simulink model "FMS"  (R2018b)
settings: configuration reference "fms_config" (kept outside this file)
values from neighbouring files (symbols this model uses):
  FMS_EXPORT = Simulink.Parameter(FMS_EXPORT_VALUE)    [fms_model_init.m]
  FMS_PARAM = Simulink.Parameter(FMS_PARAM_VALUE)    [fms_model_init.m]
undefined symbols (not defined in the file or in its folder): actuator_cmd, ay_cmd, cmd_mask, ControlMode, ctrl_mode, DiscIntNeverNeededParam, FMS_Cmd, mode, PilotMode, r_cmd, reset, state, status, theta_cmd, timestamp, u_cmd, VehicleState, VehicleStatus, w_cmd, wp_consume, wp_current
libraries: simulink x27, FMT_Model_Lib x21, hdlsllib x4
(part 2 of 3)

== system FMS/FMS Commander/Commander/Arm/Assist/Position/Altitude Command/Detect Movement ==
  FMS_In : Inport
  Abs : Abs
  Abs1 : Abs
  Bus Selector : BusSelector  OutputSignals=Pilot_Cmd.stick_throttle,INS_Out.vd
  Compare To Constant : simulink/Logic and Bit Operations/Compare To Constant  relop=>  const=FMS_PARAM.THROTTLE_DZ  OutDataTypeStr=boolean
  Motion Status : Stateflow chart  TreatAsAtomicUnit=on
  motion_state : Outport
  wires:
  FMS_In/1 -> Bus Selector/1
  Abs1/1 -> Compare To Constant/1
  Motion Status/1(state) -> motion_state/1
  Compare To Constant/1 -> Motion Status/1(motion_req)
  Abs/1 -> Motion Status/2(speed)
  Bus Selector/1 -> Abs1/1  "<stick_throttle>"
  Bus Selector/2 -> Abs/1  "<vd>"

== system FMS/FMS Commander/Commander/Arm/Assist/Position/Heading Command/DeadZone2 ==
  u : Inport
  Dead Zone : DeadZone  LowerValue=-th  UpperValue=th  SaturateOnIntegerOverflow=on
  Gain : Gain  Gain=1/(1-th)
  y : Outport
  wires:
  u/1 -> Dead Zone/1
  Dead Zone/1 -> Gain/1
  Gain/1 -> y/1

== system FMS/FMS Commander/Commander/Arm/Assist/Position/Speed Command/Controller ==
  motion_state : Inport
  In Bus Element : Inport  Port=2  PortName=FMS_In
  In Bus Element1 : Inport  Port=2  PortName=FMS_In
  Brake Control : Subsystem  TreatAsAtomicUnit=on
  Hold Control : Subsystem  TreatAsAtomicUnit=on
  Merge : Merge  Inputs=3
  Move Control : Subsystem  TreatAsAtomicUnit=on
  Saturation1 : Saturate  UpperLimit=FMS_PARAM.VEL_X_LIM  LowerLimit=-FMS_PARAM.VEL_X_LIM
  Switch Case : SwitchCase  CaseConditions={MotionState.Hold, MotionState.Brake, MotionState.Move}  ShowDefaultCase=off
  uv_cmd_mPs : Outport
  wires:
  Move Control/1(uv_cmd_mPs) -> Merge/3
  Brake Control/1(u_cmd_mPs) -> Merge/2
  Hold Control/1(u_cmd_mPs) -> Merge/1
  In Bus Element/1 -> Hold Control/1(FMS_In)
  Switch Case/3 -> Move Control/Action
  Switch Case/2 -> Brake Control/Action
  Switch Case/1 -> Hold Control/Action
  motion_state/1 -> Switch Case/1
  Saturation1/1 -> uv_cmd_mPs/1
  Merge/1 -> Saturation1/1
  In Bus Element1/1 -> Move Control/1(FMS_In)

== system FMS/FMS Commander/Commander/Arm/Assist/Position/Speed Command/Detect Movement ==
  FMS_In : Inport
  Abs2 : Abs
  Bus Selector1 : BusSelector  OutputSignals=Pilot_Cmd.stick_pitch,INS_Out
  Bus_Select : Subsystem
  Compare To Constant1 : simulink/Logic and Bit Operations/Compare To Constant  relop=>  const=FMS_PARAM.PITCH_DZ  OutDataTypeStr=boolean
  Motion State : Stateflow chart  TreatAsAtomicUnit=on
  motion_state : Outport
  wires:
  FMS_In/1 -> Bus Selector1/1
  Compare To Constant1/1 -> Motion State/1(motion_req)
  Abs2/1 -> Compare To Constant1/1
  Motion State/1(state) -> motion_state/1  "pos_ms"
  Bus_Select/1(u_est_B_mPs) -> Motion State/2(speed)
  Bus Selector1/1 -> Abs2/1  "<stick_pitch>"
  Bus Selector1/2 -> Bus_Select/1(INS_Out)  "<INS_Out>"

== system FMS/FMS Commander/Commander/Arm/Assist/Stabilize/Altitude Command /DeadZone2 ==
  u : Inport
  Dead Zone : DeadZone  LowerValue=-th  UpperValue=th  SaturateOnIntegerOverflow=on
  Gain : Gain  Gain=1/(1-th)
  y : Outport
  wires:
  u/1 -> Dead Zone/1
  Dead Zone/1 -> Gain/1
  Gain/1 -> y/1

== system FMS/FMS Commander/Commander/Arm/Assist/Stabilize/Heading Command/DeadZone2 ==
  u : Inport
  Dead Zone : DeadZone  LowerValue=-th  UpperValue=th  SaturateOnIntegerOverflow=on
  Gain : Gain  Gain=1/(1-th)
  y : Outport
  wires:
  u/1 -> Dead Zone/1
  Dead Zone/1 -> Gain/1
  Gain/1 -> y/1

== system FMS/FMS Commander/Commander/Arm/Assist/Stabilize/Speed Command/DeadZone2 ==
  u : Inport
  Dead Zone : DeadZone  LowerValue=-th  UpperValue=th  SaturateOnIntegerOverflow=on
  Gain : Gain  Gain=1/(1-th)
  y : Outport
  wires:
  u/1 -> Dead Zone/1
  Dead Zone/1 -> Gain/1
  Gain/1 -> y/1

== system FMS/FMS Commander/Commander/Arm/Auto/Mission/Mission_SubSystem/Altitude Control ==
  FMS_In : Inport
  Bus Selector3 : BusSelector  OutputSignals=INS_Out.h_R
  Gain : Gain  Gain=FMS_PARAM.Z_P
  Saturation1 : Saturate  UpperLimit=FMS_PARAM.VEL_Z_LIM  LowerLimit=-FMS_PARAM.VEL_Z_LIM
  Sum2 : Sum  Inputs=|+-
  Target Height : Subsystem
  w_cmd_mPs : Outport
  wires:
  FMS_In/1 -> Bus Selector3/1, Target Height/1(FMS_In)
  Bus Selector3/1 -> Sum2/1  "<h_R>"
  Sum2/1 -> Gain/1
  Gain/1 -> Saturation1/1
  Target Height/1(h_R_sp) -> Sum2/2  "h_R_sp"
  Saturation1/1 -> w_cmd_mPs/1

== system FMS/FMS Commander/Commander/Arm/Auto/Mission/Mission_SubSystem/Position Command ==
  FMS_In : Inport
  L1 : Constant  Value=FMS_PARAM.L1  OutDataTypeStr=single
  Velocity Commander : Subsystem
  Way Points : Subsystem
  r_cmd : Outport
  wires:
  FMS_In/1 -> Velocity Commander/5(FMS_In), Way Points/1(FMS_In)
  Way Points/3(p3) -> Velocity Commander/3(p3)
  Velocity Commander/1(r_cmd) -> r_cmd/1
  Way Points/1(p1) -> Velocity Commander/1(p1)
  L1/1 -> Velocity Commander/4(L1)
  Way Points/2(p2) -> Velocity Commander/2(p2)

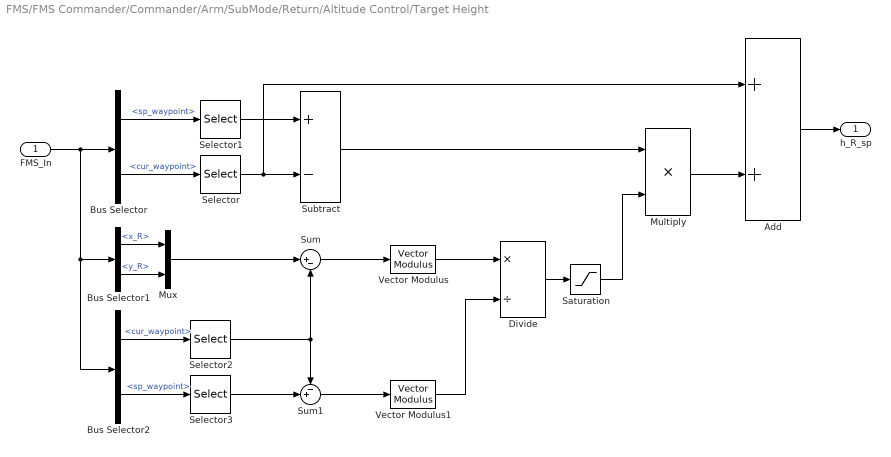
== system FMS/FMS Commander/Commander/Arm/SubMode/Return/Altitude Control/Target Height ==
  FMS_In : Inport
  Add : Sum
  Bus Selector : BusSelector  OutputSignals=Cmd_In.sp_waypoint,Cmd_In.cur_waypoint
  Bus Selector1 : BusSelector  OutputSignals=INS_Out.x_R,INS_Out.y_R
  Bus Selector2 : BusSelector  OutputSignals=Cmd_In.cur_waypoint,Cmd_In.sp_waypoint
  Divide : Product  Inputs=*/
  Multiply : Product
  Mux : Mux  Inputs=2
  Saturation : Saturate  UpperLimit=1  LowerLimit=0
  Selector : Selector  InputPortWidth=3  IndexOptions=Index vector (dialog)  Indices=3  OutputSizes=1
  Selector1 : Selector  InputPortWidth=3  IndexOptions=Index vector (dialog)  Indices=3  OutputSizes=1
  Selector2 : Selector  InputPortWidth=3  IndexOptions=Index vector (dialog)  Indices=[1 2]  OutputSizes=1
  Selector3 : Selector  InputPortWidth=3  IndexOptions=Index vector (dialog)  Indices=[1 2]  OutputSizes=1
  Subtract : Sum  Inputs=+-
  Sum : Sum  Inputs=|+-
  Sum1 : Sum  Inputs=-+|
  Vector Modulus : FMT_Model_Lib/Math/Vector Modulus
      settings: SourceProductName=FMT Toolbox
  Vector Modulus1 : FMT_Model_Lib/Math/Vector Modulus
      settings: SourceProductName=FMT Toolbox
  h_R_sp : Outport
  wires:
  Multiply/1 -> Add/2
  Bus Selector1/1 -> Mux/1  "<x_R>"
  Bus Selector/1 -> Selector1/1  "<sp_waypoint>"
  Vector Modulus1/1 -> Divide/2
  Sum1/1 -> Vector Modulus1/1
  Sum/1 -> Vector Modulus/1
  Selector2/1 -> Sum1/1, Sum/2
  FMS_In/1 -> Bus Selector2/1, Bus Selector1/1, Bus Selector/1
  Bus Selector2/2 -> Selector3/1  "<sp_waypoint>"
  Vector Modulus/1 -> Divide/1
  Bus Selector1/2 -> Mux/2  "<y_R>"
  Bus Selector2/1 -> Selector2/1  "<cur_waypoint>"
  Selector1/1 -> Subtract/1
  Mux/1 -> Sum/1
  Subtract/1 -> Multiply/1
  Divide/1 -> Saturation/1
  Selector3/1 -> Sum1/2
  Bus Selector/2 -> Selector/1  "<cur_waypoint>"
  Selector/1 -> Add/1, Subtract/2
  Saturation/1 -> Multiply/2
  Add/1 -> h_R_sp/1

== system FMS/FMS Commander/Commander/Arm/SubMode/Return/Position Command/Velocity Commander ==
  p1 : Inport
  p2 : Inport  Port=2
  p3 : Inport  Port=3
  L1 : Inport  Port=4
  In Bus Element : Inport  Port=5  PortName=FMS_In  Element=INS_Out.vn
  In Bus Element1 : Inport  Port=5  PortName=FMS_In  Element=INS_Out.ve
  AccToRate : Gain  Gain=FMS_PARAM.ACC2RATE
  L1 Reference WP : Subsystem
  Lateral Acceleration : Subsystem
  Mux1 : Mux  Inputs=2
  r_cmd : Outport
  wires:
  p3/1 -> Lateral Acceleration/3(p3), L1 Reference WP/3(P3)
  In Bus Element1/1 -> Mux1/2
  Mux1/1 -> Lateral Acceleration/1(Vg)
  p2/1 -> L1 Reference WP/2(P2)
  Lateral Acceleration/1(l1_a_cmd) -> AccToRate/1
  In Bus Element/1 -> Mux1/1
  L1 Reference WP/1(L1_WP) -> Lateral Acceleration/2(L1_WP)  "L1_WP"
  p1/1 -> L1 Reference WP/1(P1)
  L1/1 -> L1 Reference WP/4(L1), Lateral Acceleration/4(L1)
  AccToRate/1 -> r_cmd/1

== system FMS/FMS Commander/Commander/Arm/SubMode/Return/Position Command/Way Points ==
  note: P1: path start point
      | P2: path end point
      | P3: vehicle point
  FMS_In : Inport
  Bus Selector : BusSelector  OutputSignals=INS_Out.x_R,INS_Out.y_R
  Bus Selector1 : BusSelector  OutputSignals=Cmd_In.sp_waypoint
  Bus Selector2 : BusSelector  OutputSignals=Cmd_In.cur_waypoint
  Mux : Mux  Inputs=2
  Reshape : Reshape  OutputDimensionality=Customize  OutputDimensions=[2,1]
  Reshape1 : Reshape  OutputDimensionality=Customize  OutputDimensions=[2,1]
  Reshape2 : Reshape  OutputDimensionality=Customize  OutputDimensions=[2,1]
  Selector : Selector  InputPortWidth=3  IndexOptions=Index vector (dialog)  Indices=[1 2]  OutputSizes=1
  Selector1 : Selector  InputPortWidth=3  IndexOptions=Index vector (dialog)  Indices=[1 2]  OutputSizes=1
  p1 : Outport
  p2 : Outport  Port=2
  p3 : Outport  Port=3
  wires:
  Reshape2/1 -> p3/1
  Reshape1/1 -> p1/1
  Reshape/1 -> p2/1
  Bus Selector/2 -> Mux/2  "<y_R>"
  Bus Selector/1 -> Mux/1  "<x_R>"
  Mux/1 -> Reshape2/1
  FMS_In/1 -> Bus Selector2/1, Bus Selector1/1, Bus Selector/1
  Bus Selector1/1 -> Selector/1  "<sp_waypoint>"
  Selector/1 -> Reshape/1
  Bus Selector2/1 -> Selector1/1  "<cur_waypoint>"
  Selector1/1 -> Reshape1/1

== system FMS/FMS Commander/Commander/Arm/Assist/Altitude/Altitude Command/Controller/Brake Control ==
  Action Port : ActionPort  InitializeStates=reset  ActionType=case
  Brake Speed : Constant  Value=0  VectorParams1D=off  OutDataTypeStr=single
  w_cmd_mPs : Outport
  wires:
  Brake Speed/1 -> w_cmd_mPs/1

== system FMS/FMS Commander/Commander/Arm/Assist/Altitude/Altitude Command/Controller/Hold Control ==
  FMS_In : Inport
  Action Port : ActionPort  InitializeStates=reset  ActionType=case
  Bus_Selection : Subsystem
  Delay : Delay  DelayLength=1  InitialConditionSource=Input port
      settings: InputPortMap=u0,p4
  Gain2 : Gain  Gain=FMS_PARAM.Z_P  OutDataTypeStr=single
  Sum : Sum  Inputs=-+|
  w_cmd_mPs : Outport
  wires:
  FMS_In/1 -> Bus_Selection/1(FMS_In)
  Delay/1 -> Sum/2, Delay/1  "z_cmd_R"
  Sum/1 -> Gain2/1  "z_err_R"
  Bus_Selection/1(z_R_m) -> Delay/2, Sum/1  "z_est_R"
  Gain2/1 -> w_cmd_mPs/1

== system FMS/FMS Commander/Commander/Arm/Assist/Altitude/Altitude Command/Controller/Move Control ==
  FMS_In : Inport
  Action Port : ActionPort  InitializeStates=reset  ActionType=case
  Bus Selector : BusSelector  OutputSignals=Pilot_Cmd.stick_throttle
  DeadZone : Subsystem  mask{th=FMS_PARAM.THROTTLE_DZ}
      mask prompts: th "Threshold"
      mask Display: disp('Dead Zone')
  Gain1 : Gain  Gain=-FMS_PARAM.VEL_Z_LIM  OutDataTypeStr=single
  w_cmd_mPs : Outport
  wires:
  DeadZone/1(y) -> Gain1/1
  Bus Selector/1 -> DeadZone/1(u)  "<stick_throttle>"
  FMS_In/1 -> Bus Selector/1
  Gain1/1 -> w_cmd_mPs/1

== system FMS/FMS Commander/Commander/Arm/Assist/Position/Altitude Command/Controller/Brake Control ==
  Action Port : ActionPort  InitializeStates=reset  ActionType=case
  Brake Speed : Constant  Value=0  VectorParams1D=off  OutDataTypeStr=single
  w_cmd_mPs : Outport
  wires:
  Brake Speed/1 -> w_cmd_mPs/1

== system FMS/FMS Commander/Commander/Arm/Assist/Position/Altitude Command/Controller/Hold Control ==
  FMS_In : Inport
  Action Port : ActionPort  InitializeStates=reset  ActionType=case
  Bus_Selection : Subsystem
  Delay : Delay  DelayLength=1  InitialConditionSource=Input port
      settings: InputPortMap=u0,p4
  Gain2 : Gain  Gain=FMS_PARAM.Z_P  OutDataTypeStr=single
  Sum : Sum  Inputs=-+|
  w_cmd_mPs : Outport
  wires:
  FMS_In/1 -> Bus_Selection/1(FMS_In)
  Delay/1 -> Sum/2, Delay/1  "z_cmd_R"
  Sum/1 -> Gain2/1  "z_err_R"
  Bus_Selection/1(z_R_m) -> Delay/2, Sum/1  "z_est_R"
  Gain2/1 -> w_cmd_mPs/1

== system FMS/FMS Commander/Commander/Arm/Assist/Position/Altitude Command/Controller/Move Control ==
  FMS_In : Inport
  Action Port : ActionPort  InitializeStates=reset  ActionType=case
  Bus Selector : BusSelector  OutputSignals=Pilot_Cmd.stick_throttle
  DeadZone : Subsystem  mask{th=FMS_PARAM.THROTTLE_DZ}
      mask prompts: th "Threshold"
      mask Display: disp('Dead Zone')
  Gain1 : Gain  Gain=-FMS_PARAM.VEL_Z_LIM  OutDataTypeStr=single
  w_cmd_mPs : Outport
  wires:
  DeadZone/1(y) -> Gain1/1
  Bus Selector/1 -> DeadZone/1(u)  "<stick_throttle>"
  FMS_In/1 -> Bus Selector/1
  Gain1/1 -> w_cmd_mPs/1

== system FMS/FMS Commander/Commander/Arm/Assist/Position/Speed Command/Controller/Brake Control ==
  Action Port : ActionPort  InitializeStates=reset  ActionType=case
  Brake Speed : Constant  Value=0  OutDataTypeStr=single
  u_cmd_mPs : Outport
  wires:
  Brake Speed/1 -> u_cmd_mPs/1

== system FMS/FMS Commander/Commander/Arm/Assist/Position/Speed Command/Controller/Hold Control ==
  FMS_In : Inport
  Action Port : ActionPort  InitializeStates=reset  ActionType=case
  Bus Selector : BusSelector  OutputSignals=INS_Out.psi
  Bus_Selection : Subsystem
  Constant : Constant  Value=[0;0]  VectorParams1D=off  OutDataTypeStr=single
  Delay : Delay  DelayLength=1  InitialConditionSource=Input port
      settings: InputPortMap=u0,p4
  Gain2 : Gain  Gain=FMS_PARAM.X_P  OutDataTypeStr=single
  Multiply : Product  Multiplication=Matrix(*)
  Mux : Mux  Inputs=2
  Psi To DCM : FMT_Model_Lib/Transformation/Psi To DCM
      settings: SourceProductName=FMT Toolbox
  Reshape : Reshape  OutputDimensionality=Column vector (2-D)
  Selector : Selector  InputPortWidth=3  IndexOptions=Index vector (dialog)  Indices=1  OutputSizes=1
  Sum : Sum  Inputs=-+|
  u_cmd_mPs : Outport
  wires:
  Bus Selector/1 -> Psi To DCM/1  "<psi>"
  Selector/1 -> Gain2/1
  Mux/1 -> Reshape/1
  Multiply/1 -> Selector/1
  Psi To DCM/1 -> Multiply/1  "M_CO"
  Constant/1 -> Mux/2
  FMS_In/1 -> Bus_Selection/1(FMS_In), Bus Selector/1
  Delay/1 -> Sum/2, Delay/1  "x_cmd_R"
  Sum/1 -> Mux/1  "x_err_R"
  Bus_Selection/1(x_R_O_m) -> Delay/2, Sum/1  "x_est_R"
  Gain2/1 -> u_cmd_mPs/1
  Reshape/1 -> Multiply/2

== system FMS/FMS Commander/Commander/Arm/Assist/Position/Speed Command/Controller/Move Control ==
  FMS_In : Inport
  Action Port : ActionPort  InitializeStates=reset  ActionType=case
  Bus Selector : BusSelector  OutputSignals=Pilot_Cmd.stick_pitch
  DeadZone : Subsystem  mask{th=FMS_PARAM.PITCH_DZ}
      mask prompts: th "Threshold"
      mask Display: disp('Dead Zone')
  Gain6 : Gain  Gain=FMS_PARAM.VEL_X_LIM  OutDataTypeStr=single
  uv_cmd_mPs : Outport
  wires:
  Gain6/1 -> uv_cmd_mPs/1
  FMS_In/1 -> Bus Selector/1
  Bus Selector/1 -> DeadZone/1(u)  "<stick_pitch>"
  DeadZone/1(y) -> Gain6/1

== system FMS/FMS Commander/Commander/Arm/Assist/Position/Speed Command/Detect Movement/Bus_Select ==
  INS_Out : Inport
  Bus Selector1 : BusSelector  OutputSignals=vn,ve,vd
  Bus Selector2 : BusSelector  OutputSignals=quat
  Multiply : Product  Multiplication=Matrix(*)
  Mux2 : Mux  Inputs=3
  Quaternion To DCM : FMT_Model_Lib/Quaternion/Quaternion To DCM
      settings: SourceProductName=FMT Toolbox
  Selector : Selector  InputPortWidth=3  IndexOptions=Index vector (dialog)  Indices=1  OutputSizes=1
  u_est_B_mPs : Outport
  wires:
  Quaternion To DCM/1 -> Multiply/1
  Bus Selector2/1 -> Quaternion To DCM/1  "<quat>"
  Mux2/1 -> Multiply/2
  Bus Selector1/2 -> Mux2/2  "<ve>"
  Bus Selector1/1 -> Mux2/1  "<vn>"
  INS_Out/1 -> Bus Selector2/1, Bus Selector1/1
  Multiply/1 -> Selector/1
  Selector/1 -> u_est_B_mPs/1
  Bus Selector1/3 -> Mux2/3  "<vd>"

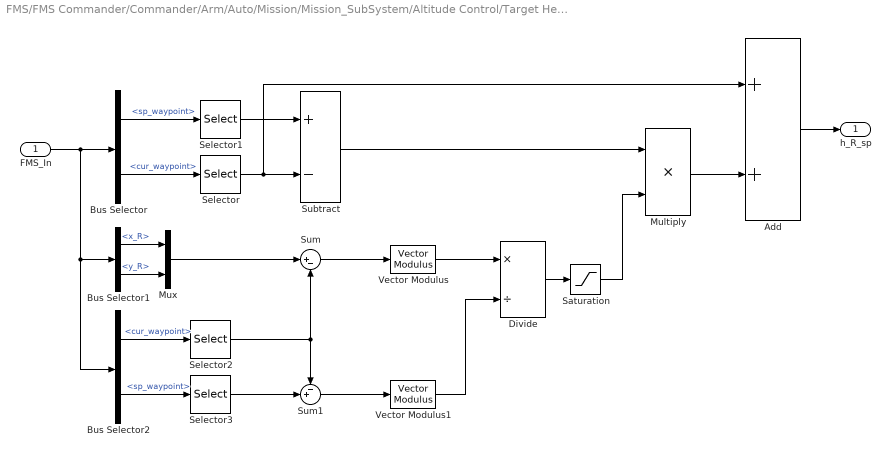
== system FMS/FMS Commander/Commander/Arm/Auto/Mission/Mission_SubSystem/Altitude Control/Target Height ==
  FMS_In : Inport
  Add : Sum
  Bus Selector : BusSelector  OutputSignals=Cmd_In.sp_waypoint,Cmd_In.cur_waypoint
  Bus Selector1 : BusSelector  OutputSignals=INS_Out.x_R,INS_Out.y_R
  Bus Selector2 : BusSelector  OutputSignals=Cmd_In.cur_waypoint,Cmd_In.sp_waypoint
  Divide : Product  Inputs=*/
  Multiply : Product
  Mux : Mux  Inputs=2
  Saturation : Saturate  UpperLimit=1  LowerLimit=0
  Selector : Selector  InputPortWidth=3  IndexOptions=Index vector (dialog)  Indices=3  OutputSizes=1
  Selector1 : Selector  InputPortWidth=3  IndexOptions=Index vector (dialog)  Indices=3  OutputSizes=1
  Selector2 : Selector  InputPortWidth=3  IndexOptions=Index vector (dialog)  Indices=[1 2]  OutputSizes=1
  Selector3 : Selector  InputPortWidth=3  IndexOptions=Index vector (dialog)  Indices=[1 2]  OutputSizes=1
  Subtract : Sum  Inputs=+-
  Sum : Sum  Inputs=|+-
  Sum1 : Sum  Inputs=-+|
  Vector Modulus : FMT_Model_Lib/Math/Vector Modulus
      settings: SourceProductName=FMT Toolbox
  Vector Modulus1 : FMT_Model_Lib/Math/Vector Modulus
      settings: SourceProductName=FMT Toolbox
  h_R_sp : Outport
  wires:
  Multiply/1 -> Add/2
  Bus Selector1/1 -> Mux/1  "<x_R>"
  Bus Selector/1 -> Selector1/1  "<sp_waypoint>"
  Vector Modulus1/1 -> Divide/2
  Sum1/1 -> Vector Modulus1/1
  Sum/1 -> Vector Modulus/1
  Selector2/1 -> Sum1/1, Sum/2
  FMS_In/1 -> Bus Selector2/1, Bus Selector1/1, Bus Selector/1
  Bus Selector2/2 -> Selector3/1  "<sp_waypoint>"
  Vector Modulus/1 -> Divide/1
  Bus Selector1/2 -> Mux/2  "<y_R>"
  Bus Selector2/1 -> Selector2/1  "<cur_waypoint>"
  Selector1/1 -> Subtract/1
  Mux/1 -> Sum/1
  Subtract/1 -> Multiply/1
  Divide/1 -> Saturation/1
  Selector3/1 -> Sum1/2
  Bus Selector/2 -> Selector/1  "<cur_waypoint>"
  Selector/1 -> Add/1, Subtract/2
  Saturation/1 -> Multiply/2
  Add/1 -> h_R_sp/1

== system FMS/FMS Commander/Commander/Arm/Auto/Mission/Mission_SubSystem/Position Command/Velocity Commander ==
  p1 : Inport
  p2 : Inport  Port=2
  p3 : Inport  Port=3
  L1 : Inport  Port=4
  In Bus Element : Inport  Port=5  PortName=FMS_In  Element=INS_Out.vn
  In Bus Element1 : Inport  Port=5  PortName=FMS_In  Element=INS_Out.ve
  AccToRate : Gain  Gain=FMS_PARAM.ACC2RATE
  L1 Reference WP : Subsystem
  Lateral Acceleration : Subsystem
  Mux1 : Mux  Inputs=2
  r_cmd : Outport
  wires:
  p3/1 -> Lateral Acceleration/3(p3), L1 Reference WP/3(P3)
  In Bus Element1/1 -> Mux1/2
  Mux1/1 -> Lateral Acceleration/1(Vg)
  p2/1 -> L1 Reference WP/2(P2)
  Lateral Acceleration/1(l1_a_cmd) -> AccToRate/1
  In Bus Element/1 -> Mux1/1
  L1 Reference WP/1(L1_WP) -> Lateral Acceleration/2(L1_WP)  "L1_WP"
  p1/1 -> L1 Reference WP/1(P1)
  L1/1 -> L1 Reference WP/4(L1), Lateral Acceleration/4(L1)
  AccToRate/1 -> r_cmd/1

== system FMS/FMS Commander/Commander/Arm/Auto/Mission/Mission_SubSystem/Position Command/Way Points ==
  note: P1: path start point
      | P2: path end point
      | P3: vehicle point
  FMS_In : Inport
  Bus Selector : BusSelector  OutputSignals=INS_Out.x_R,INS_Out.y_R
  Bus Selector1 : BusSelector  OutputSignals=Cmd_In.sp_waypoint
  Bus Selector2 : BusSelector  OutputSignals=Cmd_In.cur_waypoint
  Mux : Mux  Inputs=2
  Reshape : Reshape  OutputDimensionality=Customize  OutputDimensions=[2,1]
  Reshape1 : Reshape  OutputDimensionality=Customize  OutputDimensions=[2,1]
  Reshape2 : Reshape  OutputDimensionality=Customize  OutputDimensions=[2,1]
  Selector : Selector  InputPortWidth=3  IndexOptions=Index vector (dialog)  Indices=[1 2]  OutputSizes=1
  Selector1 : Selector  InputPortWidth=3  IndexOptions=Index vector (dialog)  Indices=[1 2]  OutputSizes=1
  p1 : Outport
  p2 : Outport  Port=2
  p3 : Outport  Port=3
  wires:
  Reshape2/1 -> p3/1
  Reshape1/1 -> p1/1
  Reshape/1 -> p2/1
  Bus Selector/2 -> Mux/2  "<y_R>"
  Bus Selector/1 -> Mux/1  "<x_R>"
  Mux/1 -> Reshape2/1
  FMS_In/1 -> Bus Selector2/1, Bus Selector1/1, Bus Selector/1
  Bus Selector1/1 -> Selector/1  "<sp_waypoint>"
  Selector/1 -> Reshape/1
  Bus Selector2/1 -> Selector1/1  "<cur_waypoint>"
  Selector1/1 -> Reshape1/1

== system FMS/FMS Commander/Commander/Arm/SubMode/Return/Position Command/Velocity Commander/L1 Reference WP ==
  P1 : Inport
  P2 : Inport  Port=2
  P3 : Inport  Port=3
  L1 : Inport  Port=4
  Compare To Constant : simulink/Logic and Bit Operations/Compare To Constant  relop=>=  const=0  OutDataTypeStr=boolean
  Compare To Constant1 : simulink/Logic and Bit Operations/Compare To Constant  relop=>  const=0  OutDataTypeStr=boolean
  NearbyRefWP : MATLAB Function  TreatAsAtomicUnit=on
  OutRegionRegWP : MATLAB Function  TreatAsAtomicUnit=on
  Reshape : Reshape  OutputDimensionality=Customize  OutputDimensions=[2,1]
  SearchL1RefWP : MATLAB Function  TreatAsAtomicUnit=on
  Switch : Switch  Criteria=u2 > Threshold
  Switch1 : Switch  Criteria=u2 > Threshold
  L1_WP : Outport
  wires:
  Reshape/1 -> L1_WP/1
  Compare To Constant/1 -> Switch/2
  NearbyRefWP/2(d) -> Compare To Constant1/1  "distance"
  SearchL1RefWP/2(u) -> Compare To Constant/1  "l1_u"
  Compare To Constant1/1 -> Switch1/2
  P1/1 -> SearchL1RefWP/1(P1), OutRegionRegWP/1(P1)
  P2/1 -> SearchL1RefWP/2(P2), NearbyRefWP/1(P2), OutRegionRegWP/2(P2)
  P3/1 -> NearbyRefWP/2(P3), SearchL1RefWP/3(P3), OutRegionRegWP/3(P3)
  Switch/1 -> Switch1/3
  L1/1 -> SearchL1RefWP/4(L1), NearbyRefWP/3(L1)
  OutRegionRegWP/1(P) -> Switch/3  "out_WP"
  Switch1/1 -> Reshape/1
  SearchL1RefWP/1(P) -> Switch/1  "L1_Ref_P"
  NearbyRefWP/1(P) -> Switch1/1  "NearbyWP"

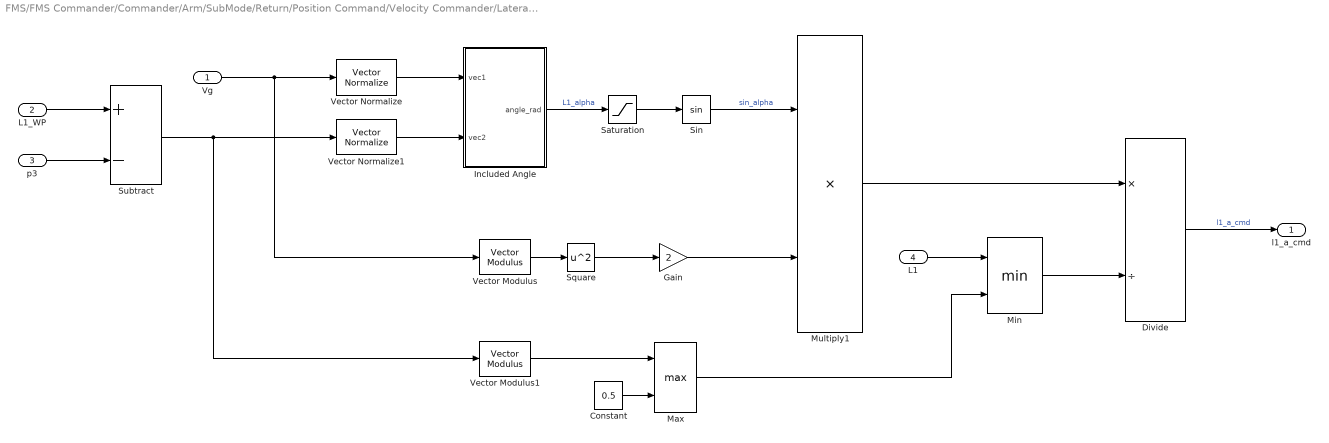
== system FMS/FMS Commander/Commander/Arm/SubMode/Return/Position Command/Velocity Commander/Lateral Acceleration ==
  Vg : Inport
  L1_WP : Inport  Port=2
  p3 : Inport  Port=3
  L1 : Inport  Port=4
  Constant : Constant  Value=0.5  OutDataTypeStr=Inherit: Inherit via back propagation
  Divide : Product  Inputs=*/
  Gain : Gain  Gain=2
  Included Angle : Subsystem
  Max : MinMax  Function=max  Inputs=2
  Min : MinMax  Inputs=2
  Multiply1 : Product
  Saturation : Saturate  UpperLimit=pi/2  LowerLimit=-pi/2
  Sin : Trigonometry
  Square : Math  Operator=square  SaturateOnIntegerOverflow=on
  Subtract : Sum  Inputs=+-
  Vector Modulus : FMT_Model_Lib/Math/Vector Modulus
      settings: SourceProductName=FMT Toolbox
  Vector Modulus1 : FMT_Model_Lib/Math/Vector Modulus
      settings: SourceProductName=FMT Toolbox
  Vector Normalize : FMT_Model_Lib/Math/Vector Normalize
      settings: SourceProductName=FMT Toolbox
  Vector Normalize1 : FMT_Model_Lib/Math/Vector Normalize
      settings: SourceProductName=FMT Toolbox
  l1_a_cmd : Outport
  wires:
  Saturation/1 -> Sin/1
  Included Angle/1(angle_rad) -> Saturation/1  "L1_alpha"
  Vector Modulus/1 -> Square/1
  Subtract/1 -> Vector Modulus1/1, Vector Normalize1/1
  Gain/1 -> Multiply1/2
  L1_WP/1 -> Subtract/1
  Vector Normalize/1 -> Included Angle/1(vec1)
  Multiply1/1 -> Divide/1
  Divide/1 -> l1_a_cmd/1  "l1_a_cmd"
  Vector Normalize1/1 -> Included Angle/2(vec2)
  Square/1 -> Gain/1
  L1/1 -> Min/1
  Vg/1 -> Vector Normalize/1, Vector Modulus/1
  Sin/1 -> Multiply1/1  "sin_alpha"
  p3/1 -> Subtract/2
  Vector Modulus1/1 -> Max/1
  Constant/1 -> Max/2
  Max/1 -> Min/2
  Min/1 -> Divide/2

== system FMS/FMS Commander/Commander/Arm/Assist/Altitude/Altitude Command/Controller/Hold Control/Bus_Selection ==
  FMS_In : Inport
  Bus Selector2 : BusSelector  OutputSignals=INS_Out.h_R
  Gain : Gain  Gain=-1
  z_R_m : Outport
  wires:
  Gain/1 -> z_R_m/1
  Bus Selector2/1 -> Gain/1  "<h_R>"
  FMS_In/1 -> Bus Selector2/1

== system FMS/FMS Commander/Commander/Arm/Assist/Altitude/Altitude Command/Controller/Move Control/DeadZone ==
  u : Inport
  Dead Zone : DeadZone  LowerValue=-th  UpperValue=th  SaturateOnIntegerOverflow=on
  Gain : Gain  Gain=1/(1-th)
  y : Outport
  wires:
  Gain/1 -> y/1
  Dead Zone/1 -> Gain/1
  u/1 -> Dead Zone/1

== system FMS/FMS Commander/Commander/Arm/Assist/Position/Altitude Command/Controller/Hold Control/Bus_Selection ==
  FMS_In : Inport
  Bus Selector2 : BusSelector  OutputSignals=INS_Out.h_R
  Gain : Gain  Gain=-1
  z_R_m : Outport
  wires:
  Gain/1 -> z_R_m/1
  Bus Selector2/1 -> Gain/1  "<h_R>"
  FMS_In/1 -> Bus Selector2/1

== system FMS/FMS Commander/Commander/Arm/Assist/Position/Altitude Command/Controller/Move Control/DeadZone ==
  u : Inport
  Dead Zone : DeadZone  LowerValue=-th  UpperValue=th  SaturateOnIntegerOverflow=on
  Gain : Gain  Gain=1/(1-th)
  y : Outport
  wires:
  Gain/1 -> y/1
  Dead Zone/1 -> Gain/1
  u/1 -> Dead Zone/1

== system FMS/FMS Commander/Commander/Arm/Assist/Position/Speed Command/Controller/Hold Control/Bus_Selection ==
  FMS_In : Inport
  Bus Selector2 : BusSelector  OutputSignals=INS_Out.x_R
  x_R_O_m : Outport
  wires:
  Bus Selector2/1 -> x_R_O_m/1  "<x_R>"
  FMS_In/1 -> Bus Selector2/1

== system FMS/FMS Commander/Commander/Arm/Assist/Position/Speed Command/Controller/Move Control/DeadZone ==
  u : Inport
  Dead Zone : DeadZone  LowerValue=-th  UpperValue=th  SaturateOnIntegerOverflow=on
  Gain : Gain  Gain=1/(1-th)
  y : Outport
  wires:
  Gain/1 -> y/1
  Dead Zone/1 -> Gain/1
  u/1 -> Dead Zone/1

== system FMS/FMS Commander/Commander/Arm/Auto/Mission/Mission_SubSystem/Position Command/Velocity Commander/L1 Reference WP ==
  P1 : Inport
  P2 : Inport  Port=2
  P3 : Inport  Port=3
  L1 : Inport  Port=4
  Compare To Constant : simulink/Logic and Bit Operations/Compare To Constant  relop=>=  const=0  OutDataTypeStr=boolean
  Compare To Constant1 : simulink/Logic and Bit Operations/Compare To Constant  relop=>  const=0  OutDataTypeStr=boolean
  NearbyRefWP : MATLAB Function  TreatAsAtomicUnit=on
  OutRegionRegWP : MATLAB Function  TreatAsAtomicUnit=on
  Reshape : Reshape  OutputDimensionality=Customize  OutputDimensions=[2,1]
  SearchL1RefWP : MATLAB Function  TreatAsAtomicUnit=on
  Switch : Switch  Criteria=u2 > Threshold
  Switch1 : Switch  Criteria=u2 > Threshold
  L1_WP : Outport
  wires:
  Reshape/1 -> L1_WP/1
  Compare To Constant/1 -> Switch/2
  NearbyRefWP/2(d) -> Compare To Constant1/1  "distance"
  SearchL1RefWP/2(u) -> Compare To Constant/1  "l1_u"
  Compare To Constant1/1 -> Switch1/2
  P1/1 -> SearchL1RefWP/1(P1), OutRegionRegWP/1(P1)
  P2/1 -> SearchL1RefWP/2(P2), NearbyRefWP/1(P2), OutRegionRegWP/2(P2)
  P3/1 -> NearbyRefWP/2(P3), SearchL1RefWP/3(P3), OutRegionRegWP/3(P3)
  Switch/1 -> Switch1/3
  L1/1 -> SearchL1RefWP/4(L1), NearbyRefWP/3(L1)
  OutRegionRegWP/1(P) -> Switch/3  "out_WP"
  Switch1/1 -> Reshape/1
  SearchL1RefWP/1(P) -> Switch/1  "L1_Ref_P"
  NearbyRefWP/1(P) -> Switch1/1  "NearbyWP"

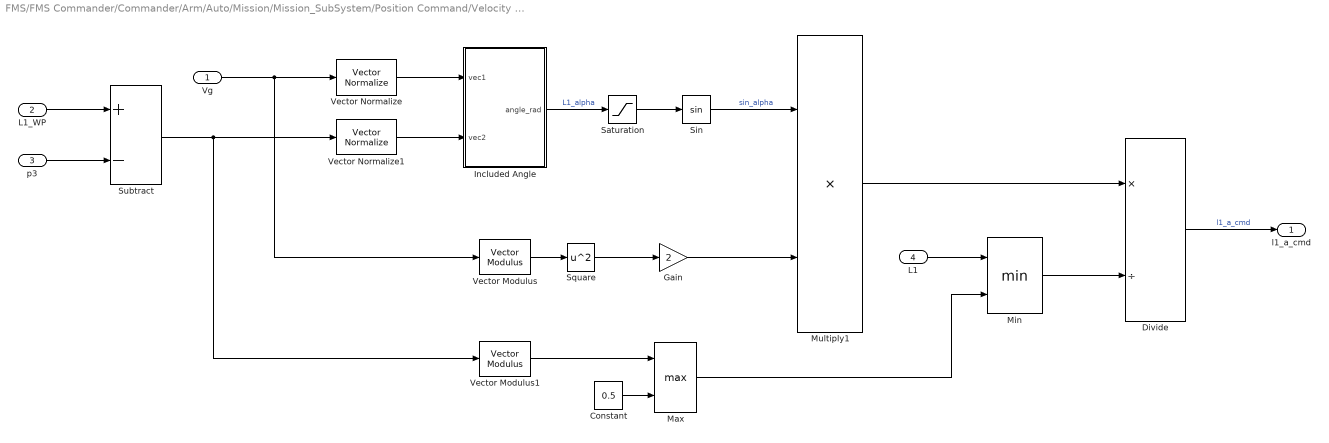
== system FMS/FMS Commander/Commander/Arm/Auto/Mission/Mission_SubSystem/Position Command/Velocity Commander/Lateral Acceleration ==
  Vg : Inport
  L1_WP : Inport  Port=2
  p3 : Inport  Port=3
  L1 : Inport  Port=4
  Constant : Constant  Value=0.5  OutDataTypeStr=Inherit: Inherit via back propagation
  Divide : Product  Inputs=*/
  Gain : Gain  Gain=2
  Included Angle : Subsystem
  Max : MinMax  Function=max  Inputs=2
  Min : MinMax  Inputs=2
  Multiply1 : Product
  Saturation : Saturate  UpperLimit=pi/2  LowerLimit=-pi/2
  Sin : Trigonometry
  Square : Math  Operator=square  SaturateOnIntegerOverflow=on
  Subtract : Sum  Inputs=+-
  Vector Modulus : FMT_Model_Lib/Math/Vector Modulus
      settings: SourceProductName=FMT Toolbox
  Vector Modulus1 : FMT_Model_Lib/Math/Vector Modulus
      settings: SourceProductName=FMT Toolbox
  Vector Normalize : FMT_Model_Lib/Math/Vector Normalize
      settings: SourceProductName=FMT Toolbox
  Vector Normalize1 : FMT_Model_Lib/Math/Vector Normalize
      settings: SourceProductName=FMT Toolbox
  l1_a_cmd : Outport
  wires:
  Saturation/1 -> Sin/1
  Included Angle/1(angle_rad) -> Saturation/1  "L1_alpha"
  Vector Modulus/1 -> Square/1
  Subtract/1 -> Vector Modulus1/1, Vector Normalize1/1
  Gain/1 -> Multiply1/2
  L1_WP/1 -> Subtract/1
  Vector Normalize/1 -> Included Angle/1(vec1)
  Multiply1/1 -> Divide/1
  Divide/1 -> l1_a_cmd/1  "l1_a_cmd"
  Vector Normalize1/1 -> Included Angle/2(vec2)
  Square/1 -> Gain/1
  L1/1 -> Min/1
  Vg/1 -> Vector Normalize/1, Vector Modulus/1
  Sin/1 -> Multiply1/1  "sin_alpha"
  p3/1 -> Subtract/2
  Vector Modulus1/1 -> Max/1
  Constant/1 -> Max/2
  Max/1 -> Min/2
  Min/1 -> Divide/2

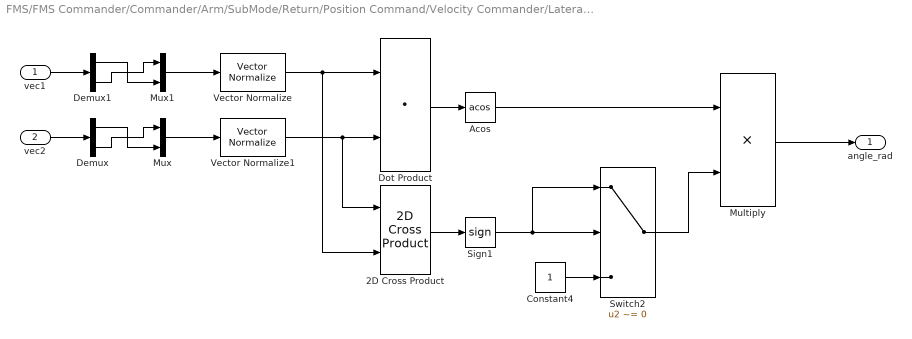
== system FMS/FMS Commander/Commander/Arm/SubMode/Return/Position Command/Velocity Commander/Lateral Acceleration/Included Angle ==
  vec1 : Inport
  vec2 : Inport  Port=2
  2D Cross Product : FMT_Model_Lib/Math/2D Cross Product
      settings: SourceProductName=FMT Toolbox
  Acos : Trigonometry  Operator=acos
  Constant4 : Constant  OutDataTypeStr=single
  Demux : Demux  Outputs=2
  Demux1 : Demux  Outputs=2
  Dot Product : DotProduct  InputSameDT=on  OutDataTypeStr=Inherit: Inherit via internal rule
  Multiply : Product
  Mux : Mux  Inputs=2
  Mux1 : Mux  Inputs=2
  Sign1 : Signum
  Switch2 : Switch  Criteria=u2 ~= 0
  Vector Normalize : FMT_Model_Lib/Math/Vector Normalize
      settings: SourceProductName=FMT Toolbox
  Vector Normalize1 : FMT_Model_Lib/Math/Vector Normalize
      settings: SourceProductName=FMT Toolbox
  angle_rad : Outport
  wires:
  Switch2/1 -> Multiply/2
  Acos/1 -> Multiply/1
  Mux/1 -> Vector Normalize1/1
  vec2/1 -> Demux/1
  Constant4/1 -> Switch2/3
  Demux/1 -> Mux/2
  vec1/1 -> Demux1/1
  Multiply/1 -> angle_rad/1
  2D Cross Product/1 -> Sign1/1
  Vector Normalize/1 -> 2D Cross Product/2, Dot Product/1
  Demux/2 -> Mux/1
  Vector Normalize1/1 -> 2D Cross Product/1, Dot Product/2
  Sign1/1 -> Switch2/2, Switch2/1
  Demux1/2 -> Mux1/1
  Mux1/1 -> Vector Normalize/1
  Demux1/1 -> Mux1/2
  Dot Product/1 -> Acos/1

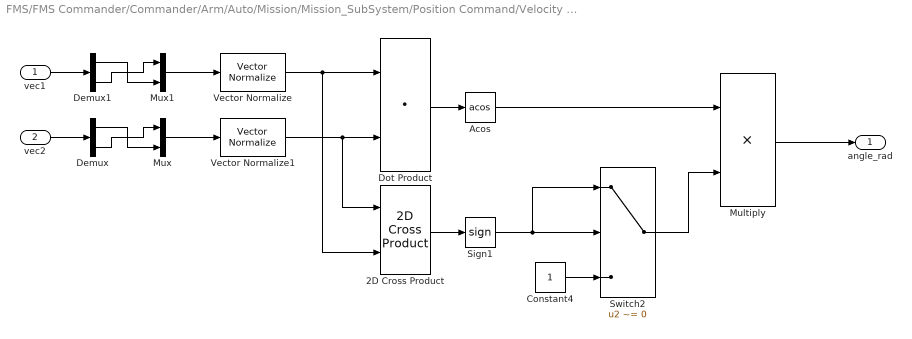
== system FMS/FMS Commander/Commander/Arm/Auto/Mission/Mission_SubSystem/Position Command/Velocity Commander/Lateral Acceleration/Included Angle ==
  vec1 : Inport
  vec2 : Inport  Port=2
  2D Cross Product : FMT_Model_Lib/Math/2D Cross Product
      settings: SourceProductName=FMT Toolbox
  Acos : Trigonometry  Operator=acos
  Constant4 : Constant  OutDataTypeStr=single
  Demux : Demux  Outputs=2
  Demux1 : Demux  Outputs=2
  Dot Product : DotProduct  InputSameDT=on  OutDataTypeStr=Inherit: Inherit via internal rule
  Multiply : Product
  Mux : Mux  Inputs=2
  Mux1 : Mux  Inputs=2
  Sign1 : Signum
  Switch2 : Switch  Criteria=u2 ~= 0
  Vector Normalize : FMT_Model_Lib/Math/Vector Normalize
      settings: SourceProductName=FMT Toolbox
  Vector Normalize1 : FMT_Model_Lib/Math/Vector Normalize
      settings: SourceProductName=FMT Toolbox
  angle_rad : Outport
  wires:
  Switch2/1 -> Multiply/2
  Acos/1 -> Multiply/1
  Mux/1 -> Vector Normalize1/1
  vec2/1 -> Demux/1
  Constant4/1 -> Switch2/3
  Demux/1 -> Mux/2
  vec1/1 -> Demux1/1
  Multiply/1 -> angle_rad/1
  2D Cross Product/1 -> Sign1/1
  Vector Normalize/1 -> 2D Cross Product/2, Dot Product/1
  Demux/2 -> Mux/1
  Vector Normalize1/1 -> 2D Cross Product/1, Dot Product/2
  Sign1/1 -> Switch2/2, Switch2/1
  Demux1/2 -> Mux1/1
  Mux1/1 -> Vector Normalize/1
  Demux1/1 -> Mux1/2
  Dot Product/1 -> Acos/1

== matlab function FMS/FMS Commander/Commander/Arm/SubMode/Return/Position Command/Velocity Commander/L1 Reference WP/NearbyRefWP ==
  data: P output; P2 input; d output; P3 input; L1 input
% Find the reference waypoint when vehicle (P3) is close to target (P2)
%
% If the vehicle is close to target (distance(P2,P3) < L1), select P2 as
% reference waypoint and return the distance, otherwise return -1.
function [P,d] = NearbyRefWP(P2, P3, L1)

P3P2 = P2 - P3;
dis = sqrt(sum(P3P2.^2));

if dis <= L1
    d = dis;
    % select P2 as reference WP
    P = P2;
else
    d = single(-1);
    % unset WP
    P = single([0; 0]);
end

== matlab function FMS/FMS Commander/Commander/Arm/SubMode/Return/Position Command/Velocity Commander/L1 Reference WP/OutRegionRegWP ==
  data: P1 input; P output; P2 input; P3 input
% Find the reference waypoint when vehicle is out of L1 region near P1P2.
%
% There are three region defined:
%   Region 1: The project point of P3 is lied on left side of P1P2
%   Region 2: The project point of P3 is lied on right side of P1P2
%   Region 3: The project point of P3 is lied on the segment line 
%
%   For the case of region 3, we select the project point as the reference
%   wayspoint. For the case of region 1, we choose P1 as reference waypoint
%   and similarly for the case of region 2, we choose P3 as reference
%   waypoint.
function P = OutRegionRefWP(P1, P2, P3)
% segment line P1P2
P1P2 = P2 - P1;
% segment line P1P3
P1P3 = P3 - P1;

% Define C as the P3 project point on line P1P2.
% Hence, P1C = dot(P1P3, P1P2)/|P1P2| * (P1P2/|P1P2|) = u * P1P2
% where u = dot(P1P3, P1P2) / |P1P2|^2.
u = dot(P1P3, P1P2) / sum(P1P2.^2);

if u <= 0
    % region 1
    P = P1;
elseif u >= 1
    % region 2
    P = P2;
else
    % region 3. C = P1C + P1
    P = u * P1P2 + P1;
end

== stateflow chart FMS/SafeMode ==
  state Other
  state Offboard
  state Mission
  state Position
  state Altitude
  state Stabilize
  (junction 21) -> Other
  Other -> (junction 68) : {target_mode = mode;}
  (junction 73) -> (junction 21) [order 2]
  (junction 68) -> (junction 78)
  (junction 73) -> Offboard [order 1] : [mode == PilotMode.Offboard]
  Offboard -> (junction 76)
  (junction 76) -> (junction 78) [order 1] : [bitget(flag, 3)&&bitget(flag, 7)&&bitget(flag, 8)]
      | {target_mode = PilotMode.Offboard;}
  (junction 1) -> (junction 73) [order 2]
  (junction 76) -> Position [order 2]
  (junction 78) -> (junction 48)
  (junction 1) -> Mission [order 1] : [mode == PilotMode.Mission]
  Mission -> (junction 16)
  (junction 16) -> (junction 48) [order 1] : [bitget(flag, 3)&&bitget(flag, 7)&&bitget(flag, 8)]
      | {target_mode = PilotMode.Mission;}
  (junction 16) -> Position [order 2]
  (junction 47) -> (junction 1) [order 2]
  (junction 48) -> (junction 51)
  (junction 47) -> Position [order 1] : [mode == PilotMode.Position]
  Position -> (junction 49)
  (junction 49) -> (junction 51) [order 1] : [bitget(flag, 3)&&bitget(flag, 7)&&bitget(flag, 8)]
      | {target_mode = PilotMode.Position;}
  (junction 55) -> (junction 47) [order 2]
  (junction 49) -> Altitude [order 2]
  (junction 51) -> (junction 2)
  (junction 55) -> Altitude [order 1] : [mode == PilotMode.Altitude]
  Altitude -> (junction 28)
  (junction 28) -> (junction 2) [order 1] : [bitget(flag, 3)&&bitget(flag, 8)]
      | {target_mode = PilotMode.Altitude;}
  (junction 24) -> (junction 55) [order 2]
  (junction 28) -> Stabilize [order 2]
  (junction 2) -> (junction 39)
  (junction 24) -> Stabilize [order 1] : [mode == PilotMode.Stabilize]
  Stabilize -> (junction 44)
  (junction 44) -> (junction 39) : [bitget(flag, 3)]{target_mode = PilotMode.Stabilize;}
  (junction 10) -> (junction 24)
  (junction 39) -> (junction 40)
  (default) -> (junction 10)
  (junction 40) -> (junction 10)
  data: target_mode output; mode input Enum: PilotMode; flag input uint32

== matlab function FMS/FMS Commander/Commander/Arm/SubMode/Return/Position Command/Velocity Commander/L1 Reference WP/SearchL1RefWP ==
  data: P1 input; P output; P2 input; P3 input; L1 input; u output
% Find reference waypoint (L1RefWP) on the line segment P1P2 which has 
% L1 distance from vehicle position (P3).
%
% The idea is to calculate the intersection point of a circle with L1 radius
% with the line segment P1P2.
%
% Define P = P1 + u * (P2 - P1), where P is the intersection point.
% Goal is calculating the u, where the valid u is between [0, 1].
%
% Input:
%   P1: start point of segment line
%   P2: start point of segment line
%   P3: circle center point, also is known as the vehicle position
%   L1: the L1 distance
% Output:
%   P: L1 reference waypoint
%   u: scale factor (valid between 0 and 1), -1 means no intersection.
function [P, u] = SearchL1RefWP(P1, P2, P3, L1)

% P1 = (x1, y1), P2 = (x2, y2), P3 = (x3, y3)
x1 = P1(1);
y1 = P1(2);
x2 = P2(1);
y2 = P2(2);
x3 = P3(1);
y3 = P3(2);

% The P is on circle and line segment, which yields:
A = (x2 - x1)^2 + (y2 - y1)^2;
B = 2 * ((x2 - x1)*(x1 - x3) + (y2 - y1)*(y1 - y3));
C = x3^2 + y3^2 + x1^2 + y1^2 - 2*(x3*x1 + y3*y1) - L1^2;
% Check root existence confition if B^2 - 4*A*C >= 0
D = B^2 - 4*A*C;
u = single(-1);
P = single([0 0]);

if D > 0
    % D>0 means we have 2 difference roots, % root is valid only if u is in range of [0, 1]
    u1 = (-B + sqrt(D)) / (2*A);
    u2 = (-B - sqrt(D)) / (2*A);
    
    if (u1>=0 && u1<=1) && (u2>=0 && u2<=1)
        % have 2 valid roots, select the one which is closer to P2 (target point)
        if u1 > u2
            u = u1; 
        else
            u = u2;
        end
    elseif (u1>=0 && u1<=1)
        % only 1 root valid, select it
        u = u1;
    elseif (u2>=0 && u2<=1)
        % only 1 root valid, select it
        u = u2;
    else
        % no valid root, which means no intersection point founded.
        return;
    end
elseif D == 0
    % D=0 means only 1 single root
    u1 = -B / (2*A);
    if (u1>=0 && u1<=1)
        % valid root, select it
        u = u1;
    else
        % no valid root, which means no intersection point founded.
        return;
    end
else
    % no valid root, which means no intersection point founded.
    return;
end

% calculate the L1 reference waypoint (P) coordinate
P(1) = x1 + u*(x2 - x1);
P(2) = y1 + u*(y2 - y1);

== stateflow chart FMS/FMS Commander/Commander/Arm/Assist/Position/Altitude Command/Detect Movement/Motion Status ==
  state Hold
    entry:
    state=MotionState.Hold;
  state Move
    entry:
    state=MotionState.Move;
  state Brake
    entry:
    state=MotionState.Brake;
  (default) -> Move
  Hold -> Move : [motion_req==1]
  Move -> Brake : [motion_req==0]
  Brake -> Move [order 2] : [motion_req==1]
  Brake -> Hold [order 1] : [speed<=0.1 || after(1.5, sec)]
  data: state output Enum: MotionState; motion_req input; speed input

== matlab function FMS/FMS Commander/Commander/Arm/Auto/Mission/Mission_SubSystem/Position Command/Velocity Commander/L1 Reference WP/NearbyRefWP ==
  data: P output; P2 input; d output; P3 input; L1 input
% Find the reference waypoint when vehicle (P3) is close to target (P2)
%
% If the vehicle is close to target (distance(P2,P3) < L1), select P2 as
% reference waypoint and return the distance, otherwise return -1.
function [P,d] = NearbyRefWP(P2, P3, L1)

P3P2 = P2 - P3;
dis = sqrt(sum(P3P2.^2));

if dis <= L1
    d = dis;
    % select P2 as reference WP
    P = P2;
else
    d = single(-1);
    % unset WP
    P = single([0; 0]);
end

== matlab function FMS/FMS Commander/Commander/Arm/Auto/Mission/Mission_SubSystem/Position Command/Velocity Commander/L1 Reference WP/OutRegionRegWP ==
  data: P1 input; P output; P2 input; P3 input
% Find the reference waypoint when vehicle is out of L1 region near P1P2.
%
% There are three region defined:
%   Region 1: The project point of P3 is lied on left side of P1P2
%   Region 2: The project point of P3 is lied on right side of P1P2
%   Region 3: The project point of P3 is lied on the segment line 
%
%   For the case of region 3, we select the project point as the reference
%   wayspoint. For the case of region 1, we choose P1 as reference waypoint
%   and similarly for the case of region 2, we choose P3 as reference
%   waypoint.
function P = OutRegionRefWP(P1, P2, P3)
% segment line P1P2
P1P2 = P2 - P1;
% segment line P1P3
P1P3 = P3 - P1;

% Define C as the P3 project point on line P1P2.
% Hence, P1C = dot(P1P3, P1P2)/|P1P2| * (P1P2/|P1P2|) = u * P1P2
% where u = dot(P1P3, P1P2) / |P1P2|^2.
u = dot(P1P3, P1P2) / sum(P1P2.^2);

if u <= 0
    % region 1
    P = P1;
elseif u >= 1
    % region 2
    P = P2;
else
    % region 3. C = P1C + P1
    P = u * P1P2 + P1;
end

== matlab function FMS/FMS Commander/Commander/Arm/Auto/Mission/Mission_SubSystem/Position Command/Velocity Commander/L1 Reference WP/SearchL1RefWP ==
  data: P1 input; P output; P2 input; P3 input; L1 input; u output
% Find reference waypoint (L1RefWP) on the line segment P1P2 which has 
% L1 distance from vehicle position (P3).
%
% The idea is to calculate the intersection point of a circle with L1 radius
% with the line segment P1P2.
%
% Define P = P1 + u * (P2 - P1), where P is the intersection point.
% Goal is calculating the u, where the valid u is between [0, 1].
%
% Input:
%   P1: start point of segment line
%   P2: start point of segment line
%   P3: circle center point, also is known as the vehicle position
%   L1: the L1 distance
% Output:
%   P: L1 reference waypoint
%   u: scale factor (valid between 0 and 1), -1 means no intersection.
function [P, u] = SearchL1RefWP(P1, P2, P3, L1)

% P1 = (x1, y1), P2 = (x2, y2), P3 = (x3, y3)
x1 = P1(1);
y1 = P1(2);
x2 = P2(1);
y2 = P2(2);
x3 = P3(1);
y3 = P3(2);

% The P is on circle and line segment, which yields:
A = (x2 - x1)^2 + (y2 - y1)^2;
B = 2 * ((x2 - x1)*(x1 - x3) + (y2 - y1)*(y1 - y3));
C = x3^2 + y3^2 + x1^2 + y1^2 - 2*(x3*x1 + y3*y1) - L1^2;
% Check root existence confition if B^2 - 4*A*C >= 0
D = B^2 - 4*A*C;
u = single(-1);
P = single([0 0]);

if D > 0
    % D>0 means we have 2 difference roots, % root is valid only if u is in range of [0, 1]
    u1 = (-B + sqrt(D)) / (2*A);
    u2 = (-B - sqrt(D)) / (2*A);
    
    if (u1>=0 && u1<=1) && (u2>=0 && u2<=1)
        % have 2 valid roots, select the one which is closer to P2 (target point)
        if u1 > u2
            u = u1; 
        else
            u = u2;
        end
    elseif (u1>=0 && u1<=1)
        % only 1 root valid, select it
        u = u1;
    elseif (u2>=0 && u2<=1)
        % only 1 root valid, select it
        u = u2;
    else
        % no valid root, which means no intersection point founded.
        return;
    end
elseif D == 0
    % D=0 means only 1 single root
    u1 = -B / (2*A);
    if (u1>=0 && u1<=1)
        % valid root, select it
        u = u1;
    else
        % no valid root, which means no intersection point founded.
        return;
    end
else
    % no valid root, which means no intersection point founded.
    return;
end

% calculate the L1 reference waypoint (P) coordinate
P(1) = x1 + u*(x2 - x1);
P(2) = y1 + u*(y2 - y1);
